simulink model "ceros_polos1"  (R2025a)
settings: Solver=VariableStepAuto  StartTime=0.0  StopTime=10.0  MaxStep=1e-2  RelTol=1e-3
values from neighbouring files (symbols this model uses):
  a = 1    [codigo_mal.m]    (also in primer_ejercicio.m = -c*d/b)
  b = 100    [codigo_mal.m]    (also in primer_ejercicio.m = (c+d)/2)
  c = 1    [codigo_mal.m]    (also in primer_ejercicio.m = -1+i)
  d = 1    [codigo_mal.m]    (also in primer_ejercicio.m = -1-i)
settings Model: Creator=fabri  LastModifiedBy=fabri

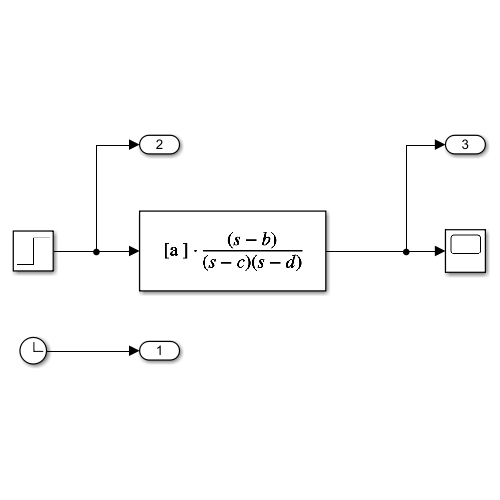
[thumbnail: Simulink's stored preview of the top-level diagram]
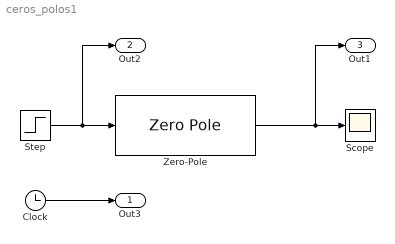
== system ceros_polos1 ==
  Clock : Clock
  Scope : Scope
      settings: ActiveDisplayYMinimum=-0.21376031532013418  ActiveDisplayYMaximum=3.4009749100625837
  Step : Step  Time=0  SampleTime=0
  Zero-Pole : ZeroPole  Zeros=[b]  Poles=[c d]  Gain=[a]
  Out3 : Outport
  Out2 : Outport  Port=2
  Out1 : Outport  Port=3
  wires:
  Step/1 -> Out2/1, Zero-Pole/1
  Zero-Pole/1 -> Out1/1, Scope/1
  Clock/1 -> Out3/1
